simulink model "testy"  (R2024a)
settings: Solver=VariableStepAuto  StartTime=0.0  StopTime=inf  RelTol=1e-3
undefined symbols (not defined in the file): dt, I_charge_max, I_max, Id_char, Imax, Ion, Iq_char, Ki_d, Ki_q, Kp_d, Kp_q, lambda, Ld, Lithium, Lq, p, Rs, Soc_max, Tmax, V_batt, Vdc_nom, Vs_max
libraries: mcbcontrolslib x4, simulink x2, spsBatteryLib x1, spsPermanentMagnetSynchronousMachineLib x1, spsSeriesRLCBranchLib x1, spsThreePhaseFaultLib x1, spsUniversalBridgeLib x1, sps_lib x1
(part 2 of 2)

== matlab function testy/Field oriented control/PIcontrol & voltage calc ==
  settings: updateMethod=DISCRETE
  data: Vd output; Id_ref input; Id input; Iq_ref input; Iq input; Vq output; Vs_max input; dt input; Kp_d input; Ki_d input; Kp_q input; Ki_q input
function [Vd, Vq] = Current_PI_control_VoltageCalc(Id_ref, Id, Iq_ref, Iq, Vs_max, dt, Kp_d, Ki_d, Kp_q, Ki_q)
%#codegen
% PI current controller with simple anti-windup and voltage magnitude limiting.
%
% Inputs:
%   Id_ref, Id, Iq_ref, Iq : currents [A]
%   Vs_max                 : max voltage magnitude (phase/space vector limit) [V]
%   dt                     : sample time [s]
%   Kp_d, Ki_d, Kp_q, Ki_q : PI gains
%
% Outputs:
%   Vd, Vq                 : dq voltage commands [V]

% Ensure scalar outputs for size inference
Vd = 0.0;
Vq = 0.0;

% Persistent integrator states
persistent int_err_Id int_err_Iq
if isempty(int_err_Id)
    int_err_Id = 0.0;
end
if isempty(int_err_Iq)
    int_err_Iq = 0.0;
end

% Anti-windup limits (axis-wise)
Vd_max = Vs_max;
Vq_max = Vs_max;

%% d-axis
err_Id = Id_ref - Id;

% integrate
int_err_Id = int_err_Id + err_Id * dt;

% PI
Vd_cmd = Kp_d * err_Id + Ki_d * int_err_Id;

% anti-windup (revert integration if saturated)
if abs(Vd_cmd) > Vd_max
    int_err_Id = int_err_Id - err_Id * dt;
    Vd_cmd = sign(Vd_cmd) * Vd_max;
end

%% q-axis
err_Iq = Iq_ref - Iq;

% integrate
int_err_Iq = int_err_Iq + err_Iq * dt;

% PI
Vq_cmd = Kp_q * err_Iq + Ki_q * int_err_Iq;

% anti-windup (revert integration if saturated)
if abs(Vq_cmd) > Vq_max
    int_err_Iq = int_err_Iq - err_Iq * dt;
    Vq_cmd = sign(Vq_cmd) * Vq_max;
end

%% Voltage limiting (vector magnitude / circle constraint)
Vs_cmd = sqrt(Vd_cmd*Vd_cmd + Vq_cmd*Vq_cmd);
if Vs_cmd > Vs_max && Vs_cmd > 1e-12
    scale = Vs_max / Vs_cmd;
    Vd_cmd = Vd_cmd * scale;
    Vq_cmd = Vq_cmd * scale;
end

Vd = Vd_cmd;
Vq = Vq_cmd;
end

== matlab function testy/Field oriented control/SVPWM algo ==
  data: v_alpha input; d_a output; v_beta input; Vdc input; apply_saturation input; d_b output; d_c output
function [d_a, d_b, d_c] = svpwm_step(v_alpha, v_beta, Vdc, apply_saturation)
% SVPWM_STEP - Space Vector PWM duty cycle generation
%
% Inputs:
%   v_alpha          : Alpha-axis voltage reference [V]
%   v_beta           : Beta-axis voltage reference [V]
%   Vdc              : DC bus voltage [V]
%   apply_saturation : 1 = scale vector to linear region, 0 = skip
%
% Outputs:
%   d_a    : Phase A duty cycle [0 to 1]
%   d_b    : Phase B duty cycle [0 to 1]
%   d_c    : Phase C duty cycle [0 to 1]
%   overmod: Overmodulation flag (1 = exceeded linear region)
%   scale  : Scaling factor applied (1.0 = no scaling)

    %% Input protection
    if Vdc <= 0
        %error('Vdc must be greater than 0');
    end

    %% Step 1 — Voltage Saturation (optional)
    v_lim = Vdc / sqrt(3);
    mag   = sqrt(v_alpha^2 + v_beta^2);

    if apply_saturation && mag > v_lim && mag > 1e-12
        scale       = v_lim / mag;
        v_alpha_use = v_alpha * scale;
        v_beta_use  = v_beta  * scale;
    else
        scale       = 1.0;
        v_alpha_use = v_alpha;
        v_beta_use  = v_beta;
    end

    %% Step 2 — Alpha-Beta to ABC (line-neutral references)
    v_a =  v_alpha_use;
    v_b = -0.5 * v_alpha_use + (sqrt(3)/2) * v_beta_use;
    v_c = -0.5 * v_alpha_use - (sqrt(3)/2) * v_beta_use;

    %% Step 3 — Zero-sequence injection (SVPWM offset)
    v_max = max([v_a, v_b, v_c]);
    v_min = min([v_a, v_b, v_c]);
    v_0   = -0.5 * (v_max + v_min);

    v_a0 = v_a + v_0;
    v_b0 = v_b + v_0;
    v_c0 = v_c + v_0;

    %% Step 4 — Duty cycle mapping
    d_a_raw = 0.5 + (v_a0 / Vdc);
    d_b_raw = 0.5 + (v_b0 / Vdc);
    d_c_raw = 0.5 + (v_c0 / Vdc);

    %% Step 6 — Clamp duties to [0, 1]
    d_a = min(max(d_a_raw, 0), 1);
    d_b = min(max(d_b_raw, 0), 1);
    d_c = min(max(d_c_raw, 0), 1);

end
